simulink model "hrg_5e_tdm_shared_readout_mismatch"  (R2025a)
settings: Solver=FixedStepDiscrete  StartTime=0.0  StopTime=c.duration  FixedStep=c.Ts  RelTol=1e-3
model workspace (MAT data in the model file):
  c.mode = 'tdm_shared'
  c.reuse = 1
  c.continuous = 0
  c.Ts = 1.83823529412e-07
  c.w = 42725.6600888
  c.omega = 0.5
  c.duration = 0.3
  c.B = 0.276990961962
  c.n = 800
  c.adcLatency = 5
  c.logDecimation = 200
  c.p.schema = 'v10.1'
  c.p.synthetic = 1
  c.p.f0 = 6800
  c.p.gamma_intrinsic = 0.712094334814
  c.p.Cs = 6e-10
  c.p.G0 = 1e-10
  c.p.kappa = 1e-06
  c.p.b = 1.1e-06
  c.p.Cds = 0
  c.p.Rs = 1000
  c.p.B = 0.276990961962
  c.p.Omega = 0.5
  c.p.Ts = 1.83823529412e-07
  c.p.Tc = 0.001
  c.p.duration = 0.3
  c.p.charge_target = 1e-11
  c.p.initial_fraction = 1
  c.p.theta0 = 0.4
  c.p.Cf = 1e-10
  c.p.Rf = 1000000000
  c.p.driver_tau = [2e-06; 2e-06]
  c.p.afe_bw = [20000; 20000]
  c.p.detect_matrix = [1  0; 0  1]
  c.p.drive_matrix = [20  0; 0  20]
  c.p.split_hz = 0.05
  c.p.stiffness_axis = 0.37
  c.p.damping_half_difference = 0
  c.p.damping_axis = -0.23
  c.p.adc_span = 2
  c.p.adc_bits = 10
  c.p.dac_span = 1
  c.p.dac_bits = 14
  c.p.vmax = 0.5
  c.p.agc_bw = 10
  c.p.quad_bw = 4
  c.p.pll_gain = 30
  c.p.max_detune = 30
  c.p.virtual_rate = 0
  c.p.virtual_start_min_s = 0.25
  c.p.virtual_settle_fraction = 0.01
  c.p.predict_heading = 1
  c.p.max_heading_rate = 100
  c.p.virtual_validated_limit = 0.2
  c.p.min_amplitude_fraction = 0.02
  c.p.min_linearity = 0.1
  c.p.max_calibration_condition = 100
  c.p.max_frame_age = 0.002
  c.p.calibrate_detection = 1
  c.p.calibrate_drive = 1
  c.p.noise_rms_V = 0
  c.p.noise_seed = 52
  c.p.carrier_hz = 6800
  c.p.Q = 30000
  c.p.pre_gain = 1
  c.p.power_gain = 20
  c.p.aaf_order = 4
  c.p.fs = 5440000
  c.p.bleed_R = 15000
  c.p.reset_tau = 2e-06
  c.p.adc_latency = 5
  c.p.log_decimation = 200
  c.p.adc_noise_rms = 0
  c.p.dac_divisor = 1
  c.p.allow_adc_underclock = 0
  c.p.seed_enabled = 0
  c.p.seed_seconds = 0.03
  c.p.seed_voltage = 0.2
  c.p.cv_mode = 'thx2024'
  c.p.thx_cv_gain = 10000
  c.p.thx_charge_per_input = 1e-06
  c.p.cv_source = 'thx2024'
  c.head.f0_Hz = 6800
  c.head.split_Hz = 0.05
  c.head.Q = 30000
  c.head.parasitic_F = 6e-10
  c.head.f_modes_Hz = [6799.975 6800.025]
  c.head.ringdown_s = 1.4043083214
  c.head.linewidth_Hz = 0.226666666667
  c.head.temperature_model = 'No per-head temperature curve supplied'
  c.head.group_shunt_F = [6e-10; 6e-10; 6e-10; 6e-10]
  c.driveEnd = 800
  c.senseStart = 1200
  c.validStart = 2000
  c.validEnd = 2800
  c.frame = 3200
  c.adcStep = 0.001953125
  c.adcMin = -1
  c.adcMax = 0.998046875
  c.dacStep = 6.103515625e-05
  c.dacMin = -0.5
  c.dacMax = 0.499938964844
  c.minEnergy = 0.0004
  c.minLinearity = 0.1
  c.agc = 62.8318530718
  c.gamma = 0.712094334814
  c.quad = 25.1327412287
  c.forceScale = 3.10732073373
  c.startCommand = [0; 0; 0; 0]
  c.seedCommand = [0; 0; -0.184212198801; -0.0778836684617]
  c.stateCount = 28
  c.pickoff = [0  0  0  0  0  0  0  0  0  0  0  0  0  0  0  0  0  0  0  0  0  0  0  0  0  0  0.1  0; 0  0  0  0  0  0  0  0  0  0  0  0  0  0  0  0  0  0  0  0  0  0  0  0  0  0  0  0.1]
  c.motion = [1  0  0  0  0  0  0  0  0  0  0  0  0  0  0  0  0  0  0  0  0  0  0  0  0  0  0  0; 0  1  0  0  0  0  0  0  0  0  0  0  0  0  0  0  0  0  0  0  0  0  0  0  0  0  0  0]
  c.electrode = [0  0  0  0  0  0  0.000213628300444  0  -0.000213628300444  0  0  0  0  0  0  0  0  0  0  0  0  0  0  0  0  0  0  0; 0  0  0  0  0  0  0  0.000213628300444  0  -0.000213628300444  0  0  0  0  0  0  0  0  0  0  0  0  0  0  0  0  0  0]
  c.cvOutputGain = 10000
  c.Ad = [0.999969157815 1.53962513641e-10 -0.00785385721515 3.93391284853e-08 -5.00204063523e-24 -2.06440054698e-29 7.59751211136e-05 -3.80429463917e-10 -7.59751211136e-05 3.80429463917e-10 0 0 ... (784 elements, 28x28)]
  c.Bd = [2.023325338e-09  5.02385057738e-17; -5.01797463451e-17  2.02332533794e-09; 7.91353351691e-07  2.62536050658e-14; -2.62152067382e-14  7.91353351649e-07; 0.0878143670381  8.50341831335e-36; 7.14438114201e-36  0.0878143670381; 3982.13043431  -2.37899750604e-16; 2.37562374806e-16  3982.13043431; -3982.13043431  2.37899750604e-16; -2.37562374806e-16  -3982.13043431; 0  0; 0  0; 0  0; 0  0; 0  0; 0  0; 0  0; 0  0; 0  0; 0  0; 0  0; 0  0; 0  0; 0  0; 0  0; 0  0; 0  0; 0  0]
  c.Af = [0.999969157815 1.53962513639e-10 -0.007853857215 3.93391284845e-08 0 0 0.00119495988637 -5.96524375398e-09 -0.00119495988637 5.96524375398e-09 0 0 ... (784 elements, 28x28)]
  c.As = [0.999969157815 1.53962513639e-10 -0.00785385721501 3.93391284846e-08 0 0 0.00108910486535 -5.43767539195e-09 -0.00108910486535 5.43767539195e-09 -0.0228351677547 -8.48854209834e-14 ... (784 elements, 28x28)]
  c.x0 = [0.921060994003; 0.389418342309; 0; 0; 0; 0; 0; 0; 0; 0; 0; 0; 0; 0; 0; 0; 0; 0; 0; 0; 0; 0; 0; 0; 0; 0; 0; 0]
  c.detect = [-2.88929518877  0  -12.1098125956  0; 0  -2.88929518877  0  -12.1098125956; 12.1098125956  0  -2.88929518877  0; 0  12.1098125956  0  -2.88929518877]
  c.drive = [0.0249909095414  0  0.00224085346117  0; 0  0.0249909095414  0  0.00224085346117; -0.00224085346117  0  0.0249909095414  0; 0  -0.00224085346117  0  0.0249909095414]
  c.gain_check.drive_pre_V_per_V = 1
  c.gain_check.sense_pre_V_per_V = 1
  c.gain_check.driver_post_gain = 20
  c.gain_check.detector_V_per_normalized_charge = 0.0803230761321
  c.gain_check.electrode_limit_V = 10
  c.gain_check.drive_modal_V_per_command = 39.8546525898
  c.gain_check.drive_condition = 1
  c.gain_check.sense_condition = 1
  c.thx_comparison.saved_Kcvd = 10000
  c.thx_comparison.saved_Kcvs = 100000
  c.thx_comparison.saved_Kcsd = 10000
  c.thx_comparison.saved_Kcss = 100000
  c.thx_comparison.matched_cv_gain = 10000
  c.thx_comparison.piezo_charge_per_input_unit_C = 1e-06
  c.thx_comparison.reuse_scope = 'THX static readout Gain, matched to drive channel source value. Piezo adapter and AAF are external.'
  c.stateRows = {'1:4', '5:6', '7:10', '11:26', '27:28'}
  c.portDriveMap = [1  0; 0  1; -1  0; 0  -1]
  c.portSenseMap = [0.5  0  -0.5  0; 0  0.5  0  -0.5]
  c.portCoupling = [1  0; 0  1; -1  0; 0  -1]
  c.portCapacitance_F = [6e-10  0  0  0; 0  6e-10  0  0; 0  0  6e-10  0; 0  0  0  6e-10]
  c.portShuntCapacitance_F = [6e-10; 6e-10; 6e-10; 6e-10]
  c.groupAngles_deg = [0; 45; 90; 135]
  c.groupNames = {'A', 'B', 'C', 'D'}
  c.commonTerminal = 'COM'
  c.portOptions.group_angles_deg = [0; 45; 90; 135]
  c.portOptions.group_charge_gain = [1; 1; 1; 1]
  c.portOptions.group_capacitance_F = [6e-10; 6e-10; 6e-10; 6e-10]
  c.portOptions.drive_on_resistance_ohm = 10
  c.portCV = [0  0  0  0  0  0  0  0  0  0  0  0  0  0  0  0  0  0  0  0  0  0  0.1  0  0  0  0  0; 0  0  0  0  0  0  0  0  0  0  0  0  0  0  0  0  0  0  0  0  0  0  0  0.1  0  0  0  0; 0  0  0  0  0  0  0  0  0  0  0  0  0  0  0  0  0  0  0  0  0  0  0  0  0.1  0  0  0; 0  0  0  0  0  0  0  0  0  0  0  0  0  0  0  0  0  0  0  0  0  0  0  0  0  0.1  0  0]
  c.readoutAnalogMismatch.readout_channel_gain = [1.01; 0.99]
  c.readoutAnalogMismatch.readout_channel_pole_Hz = [85000; 110000]
  c.readoutAnalogMismatch.readout_calibrate = 0
  c.groupVoltage = [0  0  0  0  0  0  0.000427256600888  0  0  0  0  0  0  0  0  0  0  0  0  0  0  0  0  0  0  0  0  0; 0  0  0  0  0  0  0  0.000427256600888  0  0  0  0  0  0  0  0  0  0  0  0  0  0  0  0  0  0  0  0; 0  0  0  0  0  0  0  0  0.000427256600888  0  0  0  0  0  0  0  0  0  0  0  0  0  0  0  0  0  0  0; 0  0  0  0  0  0  0  0  0  0.000427256600888  0  0  0  0  0  0  0  0  0  0  0  0  0  0  0  0  0  0]
  c.readoutCarrierResponse = [1.00357710652-0.0802861685215i; 0.986231129963-0.0609670153068i]
Description:
  | 6800 Hz whole-angle gyro. Four grouped terminals A/B/C/D relative to COM. See five_config for signed routing and physical assumptions. Native blocks only; trace columns 23:26 are the group terminal voltages.
settings Model: Creator=Administrator  LastModifiedBy=Administrator

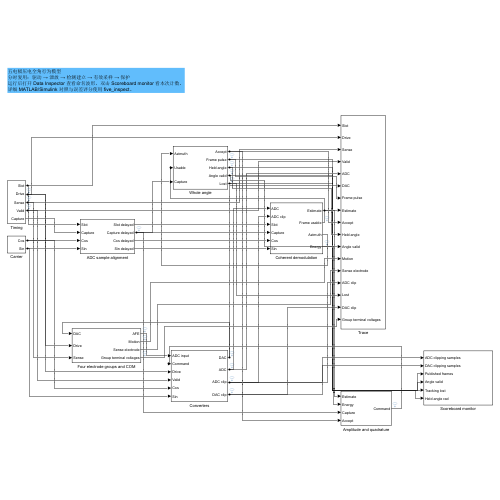
[thumbnail: Simulink's stored preview of the top-level diagram]
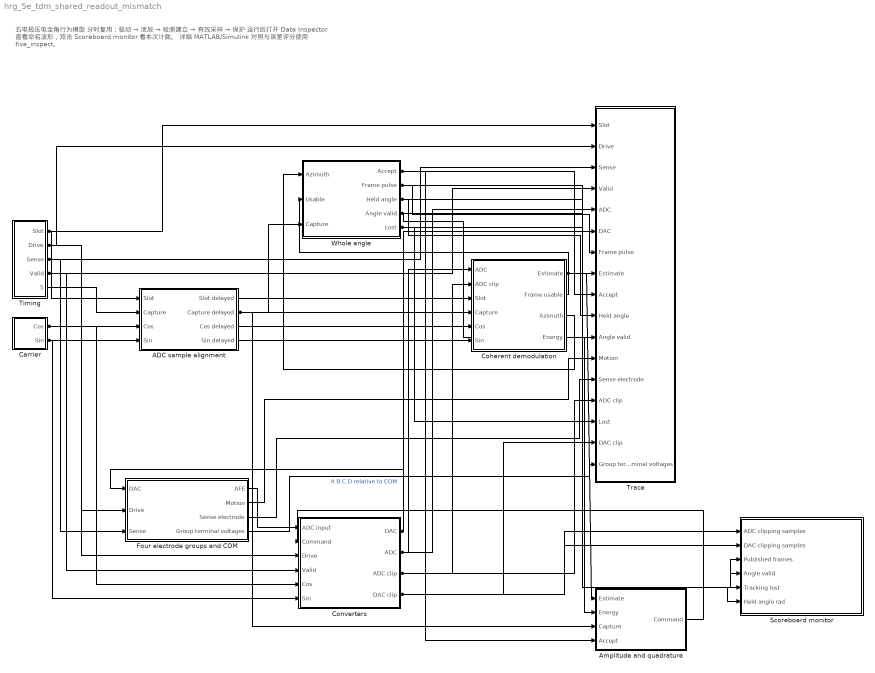
== system hrg_5e_tdm_shared_readout_mismatch ==
  note: 五电极压电全角行为模型
      | 分时复用：驱动 → 泄放 → 检测建立 → 有效采样 → 保护
      | 运行后打开 Data Inspector 查看命名波形，双击 Scoreboard monitor 看本次计数。
      | 详细 MATLAB/Simulink 对照与误差评分使用 five_inspect。
  ADC sample alignment : Subsystem
  Amplitude and quadrature : Subsystem
  Carrier : Subsystem
  Coherent demodulation : Subsystem
  Converters : Subsystem
  Four electrode groups and COM : Subsystem
  Scoreboard monitor : Subsystem
  Timing : Subsystem
  Trace : Subsystem
  Whole angle : Subsystem
  wires:
  Timing/1(Slot) -> Trace/1(Slot), ADC sample alignment/1(Slot)
  Coherent demodulation/4(Energy) -> Amplitude and quadrature/2(Energy)
  Coherent demodulation/1(Estimate) -> Amplitude and quadrature/1(Estimate), Trace/8(Estimate)
  Timing/2(Drive) -> Trace/2(Drive), Converters/3(Drive), Four electrode groups and COM/2(Drive)
  Timing/3(Sense) -> Trace/3(Sense), Four electrode groups and COM/3(Sense)
  Carrier/2(Sin) -> ADC sample alignment/4(Sin), Converters/6(Sin)
  ADC sample alignment/3(Cos delayed) -> Coherent demodulation/5(Cos)
  Carrier/1(Cos) -> Converters/5(Cos), ADC sample alignment/3(Cos)
  Converters/3(ADC clip) -> Trace/14(ADC clip), Coherent demodulation/2(ADC clip), Scoreboard monitor/1(ADC clipping samples)
  Timing/4(Valid) -> Trace/4(Valid), Converters/4(Valid)
  Amplitude and quadrature/1(Command) -> Converters/2(Command)
  ADC sample alignment/4(Sin delayed) -> Coherent demodulation/6(Sin)
  Timing/5(Capture) -> ADC sample alignment/2(Capture)
  ADC sample alignment/1(Slot delayed) -> Coherent demodulation/3(Slot)
  ADC sample alignment/2(Capture delayed) -> Coherent demodulation/4(Capture), Amplitude and quadrature/3(Capture), Whole angle/3(Capture)
  Whole angle/5(Lost) -> Trace/15(Lost), Scoreboard monitor/5(Tracking lost)
  Four electrode groups and COM/1(AFE) -> Converters/1(ADC input)
  Four electrode groups and COM/2(Motion) -> Trace/12(Motion)
  Four electrode groups and COM/3(Sense electrode) -> Trace/13(Sense electrode)
  Four electrode groups and COM/4(Group terminal voltages) -> Trace/17(Group terminal voltages)  "A B C D relative to COM"
  Converters/2(ADC) -> Trace/5(ADC), Coherent demodulation/1(ADC)
  Whole angle/1(Accept) -> Amplitude and quadrature/4(Accept), Trace/9(Accept)
  Whole angle/2(Frame pulse) -> Trace/7(Frame pulse), Scoreboard monitor/3(Published frames)
  Whole angle/3(Held angle) -> Trace/10(Held angle), Scoreboard monitor/6(Held angle rad)
  Whole angle/4(Angle valid) -> Trace/11(Angle valid), Scoreboard monitor/4(Angle valid)
  Converters/1(DAC) -> Four electrode groups and COM/1(DAC), Trace/6(DAC)
  Converters/4(DAC clip) -> Trace/16(DAC clip), Scoreboard monitor/2(DAC clipping samples)
  Coherent demodulation/2(Frame usable) -> Whole angle/2(Usable)
  Coherent demodulation/3(Azimuth) -> Whole angle/1(Azimuth)

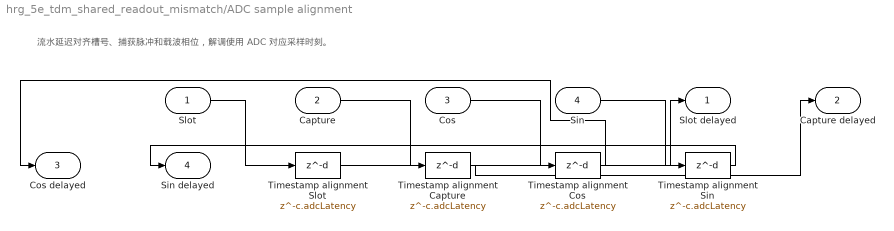
== system hrg_5e_tdm_shared_readout_mismatch/ADC sample alignment ==
  note: 流水延迟对齐槽号、捕获脉冲和载波相位，解调使用 ADC 对应采样时刻。
  Slot : Inport
  Capture : Inport  Port=2
  Cos : Inport  Port=3
  Sin : Inport  Port=4
  Timestamp alignment Capture : Delay  DelayLength=c.adcLatency  InitialCondition=0  SampleTime=c.Ts
  Timestamp alignment Cos : Delay  DelayLength=c.adcLatency  InitialCondition=0  SampleTime=c.Ts
  Timestamp alignment Sin : Delay  DelayLength=c.adcLatency  InitialCondition=0  SampleTime=c.Ts
  Timestamp alignment Slot : Delay  DelayLength=c.adcLatency  InitialCondition=-1  SampleTime=c.Ts
  Slot delayed : Outport
  Capture delayed : Outport  Port=2
  Cos delayed : Outport  Port=3
  Sin delayed : Outport  Port=4
  wires:
  Slot/1 -> Timestamp alignment Slot/1
  Timestamp alignment Slot/1 -> Slot delayed/1
  Capture/1 -> Timestamp alignment Capture/1
  Timestamp alignment Capture/1 -> Capture delayed/1
  Cos/1 -> Timestamp alignment Cos/1
  Timestamp alignment Cos/1 -> Cos delayed/1
  Sin/1 -> Timestamp alignment Sin/1
  Timestamp alignment Sin/1 -> Sin delayed/1

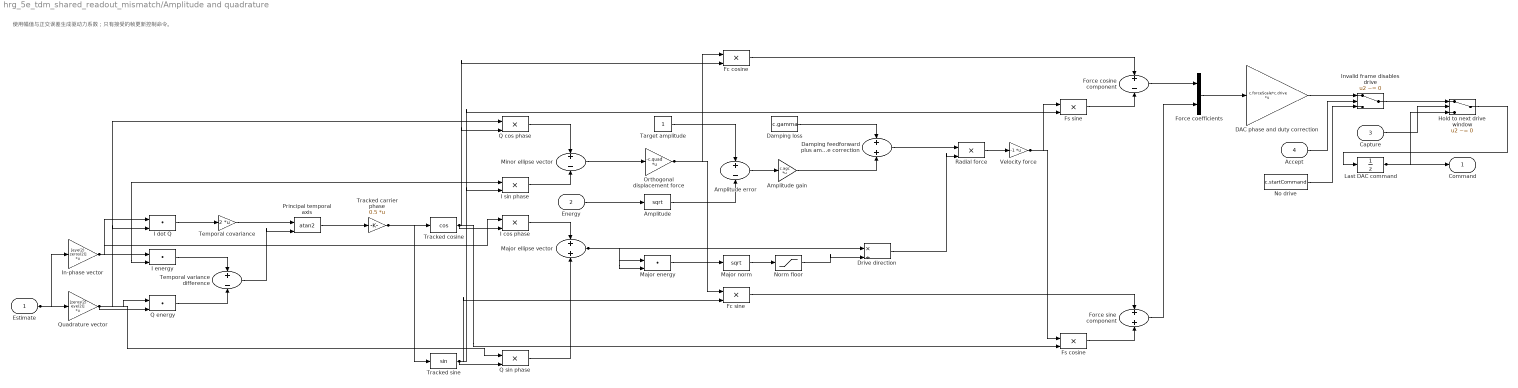
== system hrg_5e_tdm_shared_readout_mismatch/Amplitude and quadrature ==
  note: 使用幅值与正交误差生成驱动力系数；只有接受的帧更新控制命令。
  Estimate : Inport
  Energy : Inport  Port=2
  Capture : Inport  Port=3
  Accept : Inport  Port=4
  Amplitude : Sqrt
  Amplitude error : Sum  Inputs=+-
  Amplitude gain : Gain  Gain=c.agc  Multiplication=Matrix(K*u)
  DAC phase and duty correction : Gain  Gain=c.forceScale*c.drive  Multiplication=Matrix(K*u)
  Damping feedforward plus amplitude correction : Sum
  Damping loss : Constant  Value=c.gamma
  Drive direction : Product  Inputs=*/
  Fc cosine : Product
  Fc sine : Product
  Force coefficients : Mux  Inputs=2
  Force cosine component : Sum  Inputs=+-
  Force sine component : Sum
  Fs cosine : Product
  Fs sine : Product
  Hold to next drive window : Switch  Criteria=u2 ~= 0  SaturateOnIntegerOverflow=off  InputSameDT=off
  I cos phase : Product
  I dot Q : DotProduct  OutDataTypeStr=Inherit: Inherit via internal rule
  I energy : DotProduct  OutDataTypeStr=Inherit: Inherit via internal rule
  I sin phase : Product
  In-phase vector : Gain  Gain=[eye(2) zeros(2)]  Multiplication=Matrix(K*u)
  Invalid frame disables drive : Switch  Criteria=u2 ~= 0  SaturateOnIntegerOverflow=off  InputSameDT=off
  Last DAC command : UnitDelay  InitialCondition=c.startCommand  SampleTime=c.Ts  HasFrameUpgradeWarning=on
  Major ellipse vector : Sum
  Major energy : DotProduct  OutDataTypeStr=Inherit: Inherit via internal rule
  Major norm : Sqrt
  Minor ellipse vector : Sum  Inputs=+-
  No drive : Constant  Value=c.startCommand
  Norm floor : Saturate  UpperLimit=inf  LowerLimit=1e-9
  Orthogonal displacement force : Gain  Gain=-c.quad  Multiplication=Matrix(K*u)
  Principal temporal axis : Trigonometry  Operator=atan2
  Q cos phase : Product
  Q energy : DotProduct  OutDataTypeStr=Inherit: Inherit via internal rule
  Q sin phase : Product
  Quadrature vector : Gain  Gain=[zeros(2) eye(2)]  Multiplication=Matrix(K*u)
  Radial force : Product
  Target amplitude : Constant
  Temporal covariance : Gain  Gain=2  Multiplication=Matrix(K*u)
  Temporal variance difference : Sum  Inputs=+-
  Tracked carrier phase : Gain  Gain=0.5  Multiplication=Matrix(K*u)
  Tracked cosine : Trigonometry  Operator=cos
  Tracked sine : Trigonometry
  Velocity force : Gain  Gain=-1  Multiplication=Matrix(K*u)
  Command : Outport
  wires:
  Estimate/1 -> In-phase vector/1, Quadrature vector/1
  Temporal covariance/1 -> Principal temporal axis/1
  I dot Q/1 -> Temporal covariance/1
  In-phase vector/1 -> I cos phase/1, I sin phase/1, I energy/2, I energy/1, I dot Q/1
  Tracked carrier phase/1 -> Tracked cosine/1, Tracked sine/1
  Temporal variance difference/1 -> Principal temporal axis/2
  Minor ellipse vector/1 -> Orthogonal displacement force/1
  Quadrature vector/1 -> Q sin phase/1, Q cos phase/1, Q energy/1, Q energy/2, I dot Q/2
  I energy/1 -> Temporal variance difference/1
  Q energy/1 -> Temporal variance difference/2
  Principal temporal axis/1 -> Tracked carrier phase/1
  Damping feedforward plus amplitude correction/1 -> Radial force/1
  Tracked cosine/1 -> Fs cosine/2, I cos phase/2, Q cos phase/2, Fc cosine/2
  Tracked sine/1 -> Fs sine/2, I sin phase/2, Q sin phase/2, Fc sine/2
  No drive/1 -> Invalid frame disables drive/3
  Fs cosine/1 -> Force sine component/2
  I cos phase/1 -> Major ellipse vector/1
  Q cos phase/1 -> Minor ellipse vector/1
  I sin phase/1 -> Minor ellipse vector/2
  Q sin phase/1 -> Major ellipse vector/2
  Energy/1 -> Amplitude/1
  DAC phase and duty correction/1 -> Invalid frame disables drive/1
  Major ellipse vector/1 -> Drive direction/1, Major energy/1, Major energy/2
  Target amplitude/1 -> Amplitude error/1
  Orthogonal displacement force/1 -> Fc cosine/1, Fc sine/1
  Amplitude/1 -> Amplitude error/2
  Major energy/1 -> Major norm/1
  Fc cosine/1 -> Force cosine component/1
  Amplitude error/1 -> Amplitude gain/1
  Major norm/1 -> Norm floor/1
  Fc sine/1 -> Force sine component/1
  Damping loss/1 -> Damping feedforward plus amplitude correction/1
  Amplitude gain/1 -> Damping feedforward plus amplitude correction/2
  Norm floor/1 -> Drive direction/2
  Drive direction/1 -> Radial force/2
  Radial force/1 -> Velocity force/1
  Velocity force/1 -> Fs sine/1, Fs cosine/1
  Fs sine/1 -> Force cosine component/2
  Force cosine component/1 -> Force coefficients/1
  Force sine component/1 -> Force coefficients/2
  Force coefficients/1 -> DAC phase and duty correction/1
  Accept/1 -> Invalid frame disables drive/2
  Invalid frame disables drive/1 -> Hold to next drive window/1
  Capture/1 -> Hold to next drive window/2
  Last DAC command/1 -> Hold to next drive window/3, Command/1
  Hold to next drive window/1 -> Last DAC command/1

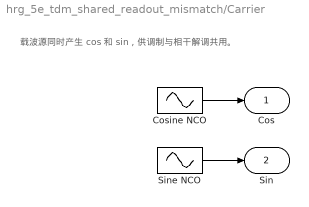
== system hrg_5e_tdm_shared_readout_mismatch/Carrier ==
  note: 载波源同时产生 cos 和 sin，供调制与相干解调共用。
  Cosine NCO : Sin  Frequency=c.w  Phase=pi/2  SampleTime=c.Ts
  Sine NCO : Sin  Frequency=c.w  SampleTime=c.Ts
  Cos : Outport
  Sin : Outport  Port=2
  wires:
  Cosine NCO/1 -> Cos/1
  Sine NCO/1 -> Sin/1

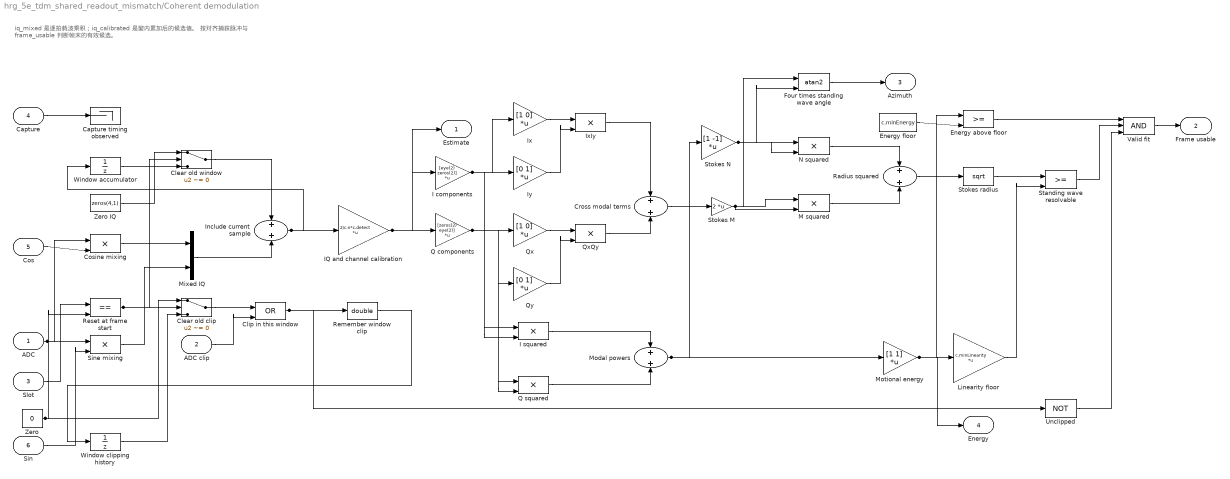
== system hrg_5e_tdm_shared_readout_mismatch/Coherent demodulation ==
  note: iq_mixed 是逐拍载波乘积；iq_calibrated 是窗内累加后的候选值。
      | 按对齐捕获脉冲与 frame_usable 判断帧末的有效候选。
  ADC : Inport
  ADC clip : Inport  Port=2
  Slot : Inport  Port=3
  Capture : Inport  Port=4
  Cos : Inport  Port=5
  Sin : Inport  Port=6
  Capture timing observed : Terminator
  Clear old clip : Switch  Criteria=u2 ~= 0  SaturateOnIntegerOverflow=off  InputSameDT=off
  Clear old window : Switch  Criteria=u2 ~= 0  SaturateOnIntegerOverflow=off  InputSameDT=off
  Clip in this window : Logic  Operator=OR  AllPortsSameDT=off  OutDataTypeStr=boolean
  Cosine mixing : Product
  Cross modal terms : Sum
  Energy above floor : RelationalOperator  OutDataTypeStr=boolean  RndMeth=Simplest  InputSameDT=off
  Energy floor : Constant  Value=c.minEnergy
  Four times standing wave angle : Trigonometry  Operator=atan2
  I components : Gain  Gain=[eye(2) zeros(2)]  Multiplication=Matrix(K*u)
  I squared : Product
  IQ and channel calibration : Gain  Gain=2/c.n*c.detect  Multiplication=Matrix(K*u)
  Include current sample : Sum
  Ix : Gain  Gain=[1 0]  Multiplication=Matrix(K*u)
  IxIy : Product
  Iy : Gain  Gain=[0 1]  Multiplication=Matrix(K*u)
  Linearity floor : Gain  Gain=c.minLinearity  Multiplication=Matrix(K*u)
  M squared : Product
  Mixed IQ : Mux  Inputs=2
  Modal powers : Sum
  Motional energy : Gain  Gain=[1 1]  Multiplication=Matrix(K*u)
  N squared : Product
  Q components : Gain  Gain=[zeros(2) eye(2)]  Multiplication=Matrix(K*u)
  Q squared : Product
  Qx : Gain  Gain=[1 0]  Multiplication=Matrix(K*u)
  QxQy : Product
  Qy : Gain  Gain=[0 1]  Multiplication=Matrix(K*u)
  Radius squared : Sum
  Remember window clip : DataTypeConversion  OutDataTypeStr=double  SaturateOnIntegerOverflow=off  RndMeth=Floor
  Reset at frame start : RelationalOperator  Operator===  OutDataTypeStr=boolean  RndMeth=Simplest  InputSameDT=off
  Sine mixing : Product
  Standing wave resolvable : RelationalOperator  OutDataTypeStr=boolean  RndMeth=Simplest  InputSameDT=off
  Stokes M : Gain  Gain=2  Multiplication=Matrix(K*u)
  Stokes N : Gain  Gain=[1 -1]  Multiplication=Matrix(K*u)
  Stokes radius : Sqrt
  Unclipped : Logic  Operator=NOT  Inputs=1  AllPortsSameDT=off  OutDataTypeStr=boolean
  Valid fit : Logic  Inputs=3  AllPortsSameDT=off  OutDataTypeStr=boolean
  Window accumulator : UnitDelay  InitialCondition=zeros(4,1)  SampleTime=c.Ts  HasFrameUpgradeWarning=on
  Window clipping history : UnitDelay  SampleTime=c.Ts  HasFrameUpgradeWarning=on
  Zero : Constant  Value=0
  Zero IQ : Constant  Value=zeros(4,1)
  Estimate : Outport
  Frame usable : Outport  Port=2
  Azimuth : Outport  Port=3
  Energy : Outport  Port=4
  wires:
  Sin/1 -> Sine mixing/2
  Cos/1 -> Cosine mixing/2
  Modal powers/1 -> Motional energy/1, Stokes N/1
  Sine mixing/1 -> Mixed IQ/2
  Capture/1 -> Capture timing observed/1
  Slot/1 -> Reset at frame start/1
  Stokes N/1 -> Four times standing wave angle/2, N squared/1, N squared/2
  ADC/1 -> Sine mixing/1, Cosine mixing/1
  Zero/1 -> Clear old clip/1, Reset at frame start/2
  Four times standing wave angle/1 -> Azimuth/1
  Window accumulator/1 -> Clear old window/3
  Unclipped/1 -> Valid fit/3
  Ix/1 -> IxIy/1
  Zero IQ/1 -> Clear old window/1
  Cosine mixing/1 -> Mixed IQ/1
  Reset at frame start/1 -> Clear old window/2, Clear old clip/2
  Window clipping history/1 -> Clear old clip/3
  Cross modal terms/1 -> Stokes M/1
  Clear old window/1 -> Include current sample/1
  Mixed IQ/1 -> Include current sample/2
  I components/1 -> I squared/1, I squared/2, Iy/1, Ix/1
  Clear old clip/1 -> Clip in this window/1
  ADC clip/1 -> Clip in this window/2
  Motional energy/1 -> Energy above floor/1, Linearity floor/1, Energy/1
  Include current sample/1 -> Window accumulator/1, IQ and channel calibration/1
  Clip in this window/1 -> Unclipped/1, Remember window clip/1
  IQ and channel calibration/1 -> I components/1, Q components/1, Estimate/1
  Remember window clip/1 -> Window clipping history/1
  Q components/1 -> Q squared/1, Q squared/2, Qx/1, Qy/1
  Iy/1 -> IxIy/2
  Qx/1 -> QxQy/1
  Linearity floor/1 -> Standing wave resolvable/2
  Qy/1 -> QxQy/2
  I squared/1 -> Modal powers/1
  Q squared/1 -> Modal powers/2
  IxIy/1 -> Cross modal terms/1
  QxQy/1 -> Cross modal terms/2
  Valid fit/1 -> Frame usable/1
  Stokes M/1 -> Four times standing wave angle/1, M squared/1, M squared/2
  N squared/1 -> Radius squared/1
  M squared/1 -> Radius squared/2
  Energy floor/1 -> Energy above floor/2
  Radius squared/1 -> Stokes radius/1
  Energy above floor/1 -> Valid fit/1
  Stokes radius/1 -> Standing wave resolvable/1
  Standing wave resolvable/1 -> Valid fit/2

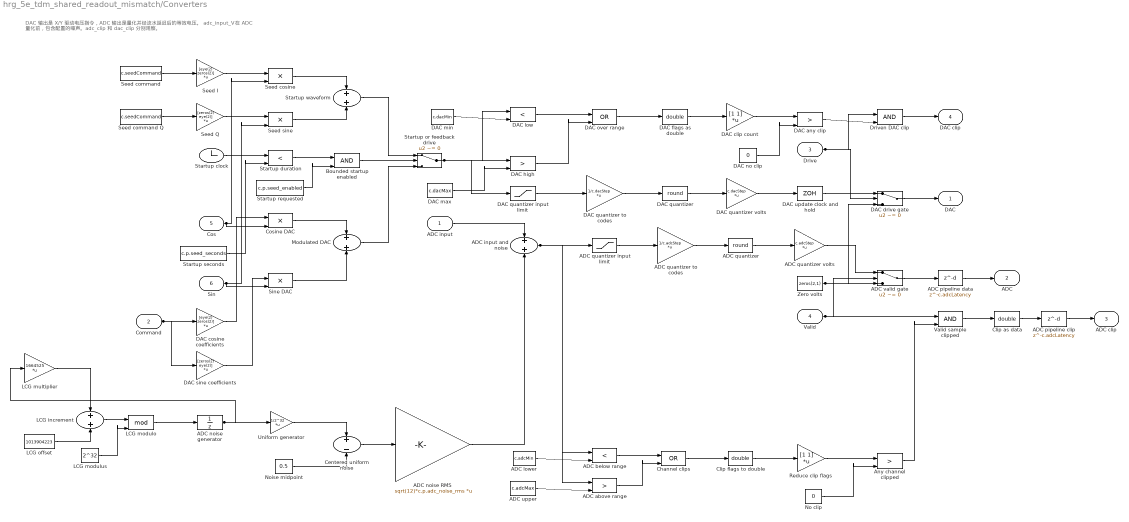
== system hrg_5e_tdm_shared_readout_mismatch/Converters ==
  note: DAC 输出是 X/Y 驱动电压指令，ADC 输出是量化并经流水延迟后的等效电压。
      | adc_input_V 在 ADC 量化前，包含配置的噪声。adc_clip 和 dac_clip 分别观察。
  ADC input : Inport
  Command : Inport  Port=2
  Drive : Inport  Port=3
  Valid : Inport  Port=4
  Cos : Inport  Port=5
  Sin : Inport  Port=6
  ADC above range : RelationalOperator  Operator=>  OutDataTypeStr=boolean  RndMeth=Simplest  InputSameDT=off
  ADC below range : RelationalOperator  Operator=<  OutDataTypeStr=boolean  RndMeth=Simplest  InputSameDT=off
  ADC input and noise : Sum
  ADC lower : Constant  Value=c.adcMin
  ADC noise RMS : Gain  Gain=sqrt(12)*c.p.adc_noise_rms  Multiplication=Matrix(K*u)
  ADC noise generator : UnitDelay  InitialCondition=[c.p.noise_seed;c.p.noise_seed+1]  SampleTime=c.Ts  HasFrameUpgradeWarning=on
  ADC pipeline clip : Delay  DelayLength=c.adcLatency  InitialCondition=0  SampleTime=c.Ts
  ADC pipeline data : Delay  DelayLength=c.adcLatency  InitialCondition=0  SampleTime=c.Ts
  ADC quantizer : Rounding  Operator=round
  ADC quantizer input limit : Saturate  UpperLimit=c.adcMax  LowerLimit=c.adcMin
  ADC quantizer to codes : Gain  Gain=1/c.adcStep  Multiplication=Matrix(K*u)
  ADC quantizer volts : Gain  Gain=c.adcStep  Multiplication=Matrix(K*u)
  ADC upper : Constant  Value=c.adcMax
  ADC valid gate : Switch  Criteria=u2 ~= 0  SaturateOnIntegerOverflow=off  InputSameDT=off
  Any channel clipped : RelationalOperator  Operator=>  OutDataTypeStr=boolean  RndMeth=Simplest  InputSameDT=off
  Bounded startup enabled : Logic  AllPortsSameDT=off  OutDataTypeStr=boolean
  Centered uniform noise : Sum  Inputs=+-
  Channel clips : Logic  Operator=OR  AllPortsSameDT=off  OutDataTypeStr=boolean
  Clip as data : DataTypeConversion  OutDataTypeStr=double  SaturateOnIntegerOverflow=off  RndMeth=Floor
  Clip flags to double : DataTypeConversion  OutDataTypeStr=double  SaturateOnIntegerOverflow=off  RndMeth=Floor
  Cosine DAC : Product
  DAC any clip : RelationalOperator  Operator=>  OutDataTypeStr=boolean  RndMeth=Simplest  InputSameDT=off
  DAC clip count : Gain  Gain=[1 1]  Multiplication=Matrix(K*u)
  DAC cosine coefficients : Gain  Gain=[eye(2) zeros(2)]  Multiplication=Matrix(K*u)
  DAC drive gate : Switch  Criteria=u2 ~= 0  SaturateOnIntegerOverflow=off  InputSameDT=off
  DAC flags as double : DataTypeConversion  OutDataTypeStr=double  SaturateOnIntegerOverflow=off  RndMeth=Floor
  DAC high : RelationalOperator  Operator=>  OutDataTypeStr=boolean  RndMeth=Simplest  InputSameDT=off
  DAC low : RelationalOperator  Operator=<  OutDataTypeStr=boolean  RndMeth=Simplest  InputSameDT=off
  DAC max : Constant  Value=c.dacMax
  DAC min : Constant  Value=c.dacMin
  DAC no clip : Constant  Value=0
  DAC over range : Logic  Operator=OR  AllPortsSameDT=off  OutDataTypeStr=boolean
  DAC quantizer : Rounding  Operator=round
  DAC quantizer input limit : Saturate  UpperLimit=c.dacMax  LowerLimit=c.dacMin
  DAC quantizer to codes : Gain  Gain=1/c.dacStep  Multiplication=Matrix(K*u)
  DAC quantizer volts : Gain  Gain=c.dacStep  Multiplication=Matrix(K*u)
  DAC sine coefficients : Gain  Gain=[zeros(2) eye(2)]  Multiplication=Matrix(K*u)
  DAC update clock and hold : ZeroOrderHold  SampleTime=c.Ts*c.p.dac_divisor
  Driven DAC clip : Logic  AllPortsSameDT=off  OutDataTypeStr=boolean
  LCG increment : Sum
  LCG modulo : Math  Operator=mod
  LCG modulus : Constant  Value=2^32
  LCG multiplier : Gain  Gain=1664525  Multiplication=Matrix(K*u)
  LCG offset : Constant  Value=1013904223
  Modulated DAC : Sum
  No clip : Constant  Value=0
  Noise midpoint : Constant  Value=0.5
  Reduce clip flags : Gain  Gain=[1 1]  Multiplication=Matrix(K*u)
  Seed I : Gain  Gain=[eye(2) zeros(2)]  Multiplication=Matrix(K*u)
  Seed Q : Gain  Gain=[zeros(2) eye(2)]  Multiplication=Matrix(K*u)
  Seed command : Constant  Value=c.seedCommand
  Seed command Q : Constant  Value=c.seedCommand
  Seed cosine : Product
  Seed sine : Product
  Sine DAC : Product
  Startup clock : Clock
  Startup duration : RelationalOperator  Operator=<  OutDataTypeStr=boolean  RndMeth=Simplest  InputSameDT=off
  Startup or feedback drive : Switch  Criteria=u2 ~= 0  SaturateOnIntegerOverflow=off  InputSameDT=off
  Startup requested : Constant  Value=c.p.seed_enabled
  Startup seconds : Constant  Value=c.p.seed_seconds
  Startup waveform : Sum
  Uniform generator : Gain  Gain=1/2^32  Multiplication=Matrix(K*u)
  Valid sample clipped : Logic  AllPortsSameDT=off  OutDataTypeStr=boolean
  Zero volts : Constant  Value=zeros(2,1)
  DAC : Outport
  ADC : Outport  Port=2
  ADC clip : Outport  Port=3
  DAC clip : Outport  Port=4
  wires:
  Seed command/1 -> Seed I/1
  Seed cosine/1 -> Startup waveform/1
  ADC quantizer volts/1 -> ADC valid gate/1
  Startup requested/1 -> Bounded startup enabled/2
  LCG multiplier/1 -> LCG increment/1
  Channel clips/1 -> Clip flags to double/1
  Startup or feedback drive/1 -> DAC quantizer input limit/1, DAC low/1, DAC high/1
  LCG modulus/1 -> LCG modulo/2
  LCG offset/1 -> LCG increment/2
  Reduce clip flags/1 -> Any channel clipped/1
  Cos/1 -> Cosine DAC/2, Seed cosine/2
  LCG increment/1 -> LCG modulo/1
  Bounded startup enabled/1 -> Startup or feedback drive/2
  ADC below range/1 -> Channel clips/1
  Seed command Q/1 -> Seed Q/1
  LCG modulo/1 -> ADC noise generator/1
  Command/1 -> DAC sine coefficients/1, DAC cosine coefficients/1
  ADC input/1 -> ADC input and noise/1
  Seed I/1 -> Seed cosine/1
  Seed Q/1 -> Seed sine/1
  Startup clock/1 -> Startup duration/1
  Startup seconds/1 -> Startup duration/2
  Sin/1 -> Sine DAC/2, Seed sine/2
  ADC quantizer/1 -> ADC quantizer volts/1
  DAC cosine coefficients/1 -> Cosine DAC/1
  DAC sine coefficients/1 -> Sine DAC/1
  DAC min/1 -> DAC low/2
  ADC noise generator/1 -> LCG multiplier/1, Uniform generator/1
  Seed sine/1 -> Startup waveform/2
  ADC quantizer input limit/1 -> ADC quantizer to codes/1
  Startup duration/1 -> Bounded startup enabled/1
  Cosine DAC/1 -> Modulated DAC/1
  No clip/1 -> Any channel clipped/2
  Sine DAC/1 -> Modulated DAC/2
  DAC quantizer volts/1 -> DAC update clock and hold/1
  ADC pipeline data/1 -> ADC/1
  DAC flags as double/1 -> DAC clip count/1
  ADC above range/1 -> Channel clips/2
  Uniform generator/1 -> Centered uniform noise/1
  ADC quantizer to codes/1 -> ADC quantizer/1
  Noise midpoint/1 -> Centered uniform noise/2
  Startup waveform/1 -> Startup or feedback drive/1
  ADC noise RMS/1 -> ADC input and noise/2
  Modulated DAC/1 -> Startup or feedback drive/3
  Centered uniform noise/1 -> ADC noise RMS/1
  DAC max/1 -> DAC high/2
  DAC low/1 -> DAC over range/1
  DAC high/1 -> DAC over range/2
  DAC clip count/1 -> DAC any clip/1
  DAC quantizer input limit/1 -> DAC quantizer to codes/1
  ADC input and noise/1 -> ADC below range/1, ADC quantizer input limit/1, ADC above range/1
  ADC lower/1 -> ADC below range/2
  Zero volts/1 -> DAC drive gate/3, ADC valid gate/3
  Drive/1 -> DAC drive gate/2, Driven DAC clip/1
  ADC upper/1 -> ADC above range/2
  DAC over range/1 -> DAC flags as double/1
  DAC quantizer to codes/1 -> DAC quantizer/1
  DAC quantizer/1 -> DAC quantizer volts/1
  DAC no clip/1 -> DAC any clip/2
  Clip flags to double/1 -> Reduce clip flags/1
  DAC any clip/1 -> Driven DAC clip/2
  DAC update clock and hold/1 -> DAC drive gate/1
  Driven DAC clip/1 -> DAC clip/1
  Valid/1 -> Valid sample clipped/1, ADC valid gate/2
  DAC drive gate/1 -> DAC/1
  ADC valid gate/1 -> ADC pipeline data/1
  Any channel clipped/1 -> Valid sample clipped/2
  Valid sample clipped/1 -> Clip as data/1
  Clip as data/1 -> ADC pipeline clip/1
  ADC pipeline clip/1 -> ADC clip/1

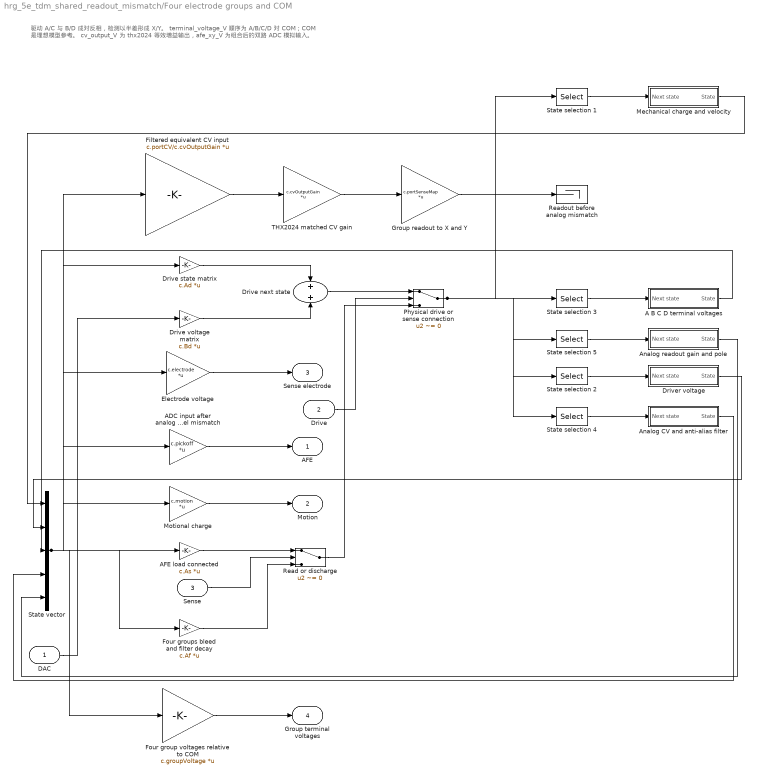
== system hrg_5e_tdm_shared_readout_mismatch/Four electrode groups and COM ==
  note: 驱动 A/C 与 B/D 成对反相，检测以半差形成 X/Y。
      | terminal_voltage_V 顺序为 A/B/C/D 对 COM；COM 是理想模型参考。
      | cv_output_V 为 thx2024 等效增益输出，afe_xy_V 为组合后的双路 ADC 模拟输入。
  DAC : Inport
  Drive : Inport  Port=2
  Sense : Inport  Port=3
  A B C D terminal voltages : Subsystem
  ADC input after analog channel mismatch : Gain  Gain=c.pickoff  Multiplication=Matrix(K*u)
  AFE load connected : Gain  Gain=c.As  Multiplication=Matrix(K*u)
  Analog CV and anti-alias filter : Subsystem
  Analog readout gain and pole : Subsystem
  Drive next state : Sum
  Drive state matrix : Gain  Gain=c.Ad  Multiplication=Matrix(K*u)
  Drive voltage matrix : Gain  Gain=c.Bd  Multiplication=Matrix(K*u)
  Driver voltage : Subsystem
  Electrode voltage : Gain  Gain=c.electrode  Multiplication=Matrix(K*u)
  Filtered equivalent CV input : Gain  Gain=c.portCV/c.cvOutputGain  Multiplication=Matrix(K*u)
  Four group voltages relative to COM : Gain  Gain=c.groupVoltage  Multiplication=Matrix(K*u)
  Four groups bleed and filter decay : Gain  Gain=c.Af  Multiplication=Matrix(K*u)
  Group readout to X and Y : Gain  Gain=c.portSenseMap  Multiplication=Matrix(K*u)
  Mechanical charge and velocity : Subsystem
  Motional charge : Gain  Gain=c.motion  Multiplication=Matrix(K*u)
  Physical drive or sense connection : Switch  Criteria=u2 ~= 0  SaturateOnIntegerOverflow=off  InputSameDT=off
  Read or discharge : Switch  Criteria=u2 ~= 0  SaturateOnIntegerOverflow=off  InputSameDT=off
  Readout before analog mismatch : Terminator
  State selection 1 : Selector  InputPortWidth=28  IndexOptions=Index vector (dialog)  Indices=1:4  OutputSizes=1
  State selection 2 : Selector  InputPortWidth=28  IndexOptions=Index vector (dialog)  Indices=5:6  OutputSizes=1
  State selection 3 : Selector  InputPortWidth=28  IndexOptions=Index vector (dialog)  Indices=7:10  OutputSizes=1
  State selection 4 : Selector  InputPortWidth=28  IndexOptions=Index vector (dialog)  Indices=11:26  OutputSizes=1
  State selection 5 : Selector  InputPortWidth=28  IndexOptions=Index vector (dialog)  Indices=27:28  OutputSizes=1
  State vector : Mux  Inputs=5
  THX2024 matched CV gain : Gain  Gain=c.cvOutputGain  Multiplication=Matrix(K*u)
  AFE : Outport
  Motion : Outport  Port=2
  Sense electrode : Outport  Port=3
  Group terminal voltages : Outport  Port=4
  wires:
  AFE load connected/1 -> Read or discharge/1
  ADC input after analog channel mismatch/1 -> AFE/1
  State vector/1 -> Drive state matrix/1, Filtered equivalent CV input/1, ADC input after analog channel mismatch/1, Motional charge/1, AFE load connected/1, Electrode voltage/1, Four group voltages relative to COM/1, Four groups bleed and filter decay/1
  Electrode voltage/1 -> Sense electrode/1
  Drive state matrix/1 -> Drive next state/1
  Sense/1 -> Read or discharge/2
  DAC/1 -> Drive voltage matrix/1
  Filtered equivalent CV input/1 -> THX2024 matched CV gain/1
  Drive voltage matrix/1 -> Drive next state/2
  Drive/1 -> Physical drive or sense connection/2
  Motional charge/1 -> Motion/1
  Four groups bleed and filter decay/1 -> Read or discharge/3
  Four group voltages relative to COM/1 -> Group terminal voltages/1
  THX2024 matched CV gain/1 -> Group readout to X and Y/1
  Group readout to X and Y/1 -> Readout before analog mismatch/1
  Drive next state/1 -> Physical drive or sense connection/1
  Read or discharge/1 -> Physical drive or sense connection/3
  Physical drive or sense connection/1 -> State selection 1/1, State selection 2/1, State selection 3/1, State selection 4/1, State selection 5/1
  State selection 1/1 -> Mechanical charge and velocity/1(Next state)
  State selection 3/1 -> A B C D terminal voltages/1(Next state)
  State selection 5/1 -> Analog readout gain and pole/1(Next state)
  A B C D terminal voltages/1(State) -> State vector/3
  State selection 2/1 -> Driver voltage/1(Next state)
  State selection 4/1 -> Analog CV and anti-alias filter/1(Next state)
  Mechanical charge and velocity/1(State) -> State vector/1
  Analog readout gain and pole/1(State) -> State vector/5
  Analog CV and anti-alias filter/1(State) -> State vector/4
  Driver voltage/1(State) -> State vector/2

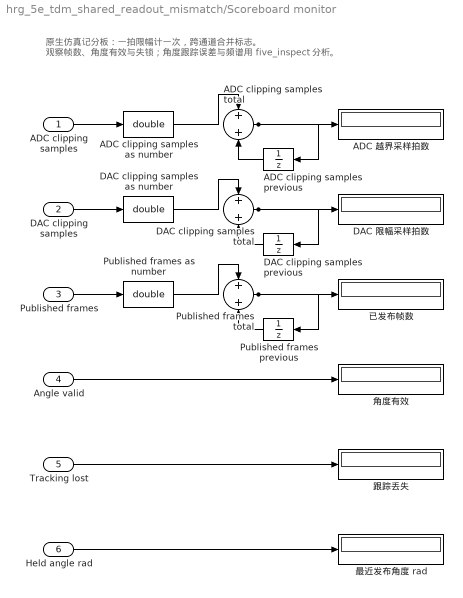
== system hrg_5e_tdm_shared_readout_mismatch/Scoreboard monitor ==
  note: 原生仿真记分板：一拍限幅计一次，跨通道合并标志。
      | 观察帧数、角度有效与失锁；角度跟踪误差与频谱用 five_inspect 分析。
  ADC clipping samples : Inport
  DAC clipping samples : Inport  Port=2
  Published frames : Inport  Port=3
  Angle valid : Inport  Port=4
  Tracking lost : Inport  Port=5
  Held angle rad : Inport  Port=6
  ADC clipping samples as number : DataTypeConversion  OutDataTypeStr=double  SaturateOnIntegerOverflow=off  RndMeth=Floor
  ADC clipping samples previous : UnitDelay  SampleTime=c.Ts  HasFrameUpgradeWarning=on
  ADC clipping samples total : Sum
  ADC 越界采样拍数 : Display
  DAC clipping samples as number : DataTypeConversion  OutDataTypeStr=double  SaturateOnIntegerOverflow=off  RndMeth=Floor
  DAC clipping samples previous : UnitDelay  SampleTime=c.Ts  HasFrameUpgradeWarning=on
  DAC clipping samples total : Sum
  DAC 限幅采样拍数 : Display
  Published frames as number : DataTypeConversion  OutDataTypeStr=double  SaturateOnIntegerOverflow=off  RndMeth=Floor
  Published frames previous : UnitDelay  SampleTime=c.Ts  HasFrameUpgradeWarning=on
  Published frames total : Sum
  已发布帧数 : Display
  最近发布角度 rad : Display
  角度有效 : Display
  跟踪丢失 : Display
  wires:
  ADC clipping samples/1 -> ADC clipping samples as number/1
  ADC clipping samples as number/1 -> ADC clipping samples total/1
  ADC clipping samples total/1 -> ADC clipping samples previous/1, ADC 越界采样拍数/1
  ADC clipping samples previous/1 -> ADC clipping samples total/2
  DAC clipping samples/1 -> DAC clipping samples as number/1
  DAC clipping samples as number/1 -> DAC clipping samples total/1
  DAC clipping samples total/1 -> DAC clipping samples previous/1, DAC 限幅采样拍数/1
  DAC clipping samples previous/1 -> DAC clipping samples total/2
  Published frames/1 -> Published frames as number/1
  Published frames as number/1 -> Published frames total/1
  Published frames total/1 -> Published frames previous/1, 已发布帧数/1
  Published frames previous/1 -> Published frames total/2
  Angle valid/1 -> 角度有效/1
  Tracking lost/1 -> 跟踪丢失/1
  Held angle rad/1 -> 最近发布角度 rad/1

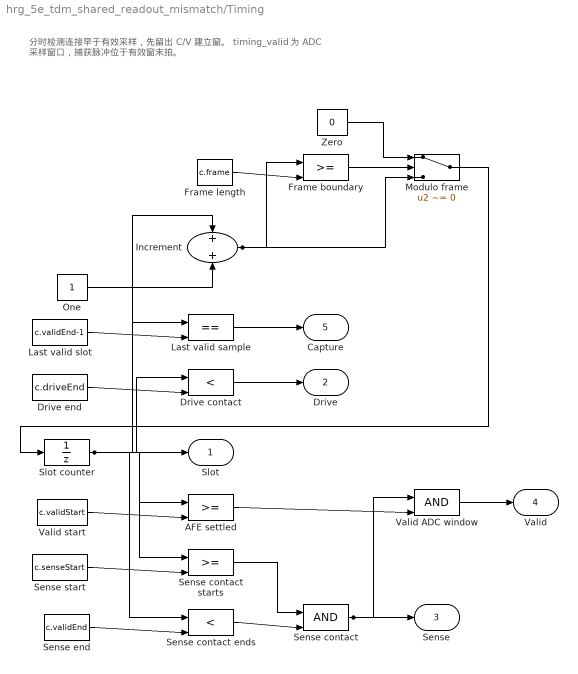
== system hrg_5e_tdm_shared_readout_mismatch/Timing ==
  note: 分时检测连接早于有效采样，先留出 C/V 建立窗。
      | timing_valid 为 ADC 采样窗口，捕获脉冲位于有效窗末拍。
  AFE settled : RelationalOperator  OutDataTypeStr=boolean  RndMeth=Simplest  InputSameDT=off
  Drive contact : RelationalOperator  Operator=<  OutDataTypeStr=boolean  RndMeth=Simplest  InputSameDT=off
  Drive end : Constant  Value=c.driveEnd
  Frame boundary : RelationalOperator  OutDataTypeStr=boolean  RndMeth=Simplest  InputSameDT=off
  Frame length : Constant  Value=c.frame
  Increment : Sum
  Last valid sample : RelationalOperator  Operator===  OutDataTypeStr=boolean  RndMeth=Simplest  InputSameDT=off
  Last valid slot : Constant  Value=c.validEnd-1
  Modulo frame : Switch  Criteria=u2 ~= 0  SaturateOnIntegerOverflow=off  InputSameDT=off
  One : Constant
  Sense contact : Logic  AllPortsSameDT=off  OutDataTypeStr=boolean
  Sense contact ends : RelationalOperator  Operator=<  OutDataTypeStr=boolean  RndMeth=Simplest  InputSameDT=off
  Sense contact starts : RelationalOperator  OutDataTypeStr=boolean  RndMeth=Simplest  InputSameDT=off
  Sense end : Constant  Value=c.validEnd
  Sense start : Constant  Value=c.senseStart
  Slot counter : UnitDelay  SampleTime=c.Ts  HasFrameUpgradeWarning=on
  Valid ADC window : Logic  AllPortsSameDT=off  OutDataTypeStr=boolean
  Valid start : Constant  Value=c.validStart
  Zero : Constant  Value=0
  Slot : Outport
  Drive : Outport  Port=2
  Sense : Outport  Port=3
  Valid : Outport  Port=4
  Capture : Outport  Port=5
  wires:
  One/1 -> Increment/2
  Last valid slot/1 -> Last valid sample/2
  Drive end/1 -> Drive contact/2
  Frame length/1 -> Frame boundary/2
  Slot counter/1 -> Drive contact/1, Sense contact starts/1, Increment/1, Last valid sample/1, Slot/1, AFE settled/1, Sense contact ends/1
  Valid start/1 -> AFE settled/2
  Last valid sample/1 -> Capture/1
  Sense end/1 -> Sense contact ends/2
  Sense start/1 -> Sense contact starts/2
  Increment/1 -> Modulo frame/3, Frame boundary/1
  Drive contact/1 -> Drive/1
  AFE settled/1 -> Valid ADC window/2
  Sense contact starts/1 -> Sense contact/1
  Sense contact ends/1 -> Sense contact/2
  Zero/1 -> Modulo frame/1
  Frame boundary/1 -> Modulo frame/2
  Sense contact/1 -> Valid ADC window/1, Sense/1
  Valid ADC window/1 -> Valid/1
  Modulo frame/1 -> Slot counter/1

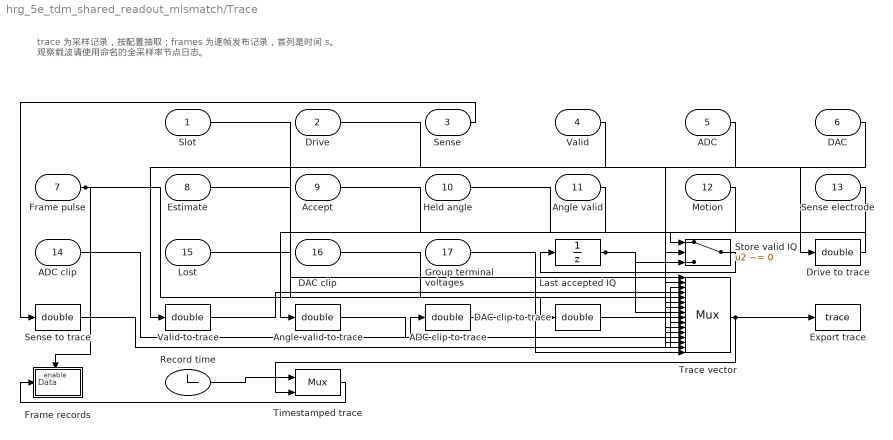
== system hrg_5e_tdm_shared_readout_mismatch/Trace ==
  note: trace 为采样记录，按配置抽取；frames 为逐帧发布记录，首列是时间 s。
      | 观察载波请使用命名的全采样率节点日志。
  Slot : Inport
  Drive : Inport  Port=2
  Sense : Inport  Port=3
  Valid : Inport  Port=4
  ADC : Inport  Port=5
  DAC : Inport  Port=6
  Frame pulse : Inport  Port=7
  Estimate : Inport  Port=8
  Accept : Inport  Port=9
  Held angle : Inport  Port=10
  Angle valid : Inport  Port=11
  Motion : Inport  Port=12
  Sense electrode : Inport  Port=13
  ADC clip : Inport  Port=14
  Lost : Inport  Port=15
  DAC clip : Inport  Port=16
  Group terminal voltages : Inport  Port=17
  ADC clip to trace : DataTypeConversion  OutDataTypeStr=double  SaturateOnIntegerOverflow=off  RndMeth=Floor
  Angle valid to trace : DataTypeConversion  OutDataTypeStr=double  SaturateOnIntegerOverflow=off  RndMeth=Floor
  DAC clip to trace : DataTypeConversion  OutDataTypeStr=double  SaturateOnIntegerOverflow=off  RndMeth=Floor
  Drive to trace : DataTypeConversion  OutDataTypeStr=double  SaturateOnIntegerOverflow=off  RndMeth=Floor
  Export trace : ToWorkspace  VariableName=trace  SampleTime=-1
      settings: Decimation=c.logDecimation
  Frame records : Subsystem
  Last accepted IQ : UnitDelay  InitialCondition=zeros(4,1)  SampleTime=c.Ts  HasFrameUpgradeWarning=on
  Record time : Clock
  Sense to trace : DataTypeConversion  OutDataTypeStr=double  SaturateOnIntegerOverflow=off  RndMeth=Floor
  Store valid IQ : Switch  Criteria=u2 ~= 0  SaturateOnIntegerOverflow=off  InputSameDT=off
  Timestamped trace : Mux  Inputs=2
  Trace vector : Mux  Inputs=16
  Valid to trace : DataTypeConversion  OutDataTypeStr=double  SaturateOnIntegerOverflow=off  RndMeth=Floor
  wires:
  Estimate/1 -> Store valid IQ/1
  Accept/1 -> Store valid IQ/2
  Last accepted IQ/1 -> Store valid IQ/3, Trace vector/8
  Store valid IQ/1 -> Last accepted IQ/1
  Drive/1 -> Drive to trace/1
  Sense/1 -> Sense to trace/1
  Valid/1 -> Valid to trace/1
  Angle valid/1 -> Angle valid to trace/1
  ADC clip/1 -> ADC clip to trace/1
  DAC clip/1 -> DAC clip to trace/1
  Slot/1 -> Trace vector/1
  Drive to trace/1 -> Trace vector/2
  Sense to trace/1 -> Trace vector/3
  Valid to trace/1 -> Trace vector/4
  ADC/1 -> Trace vector/5
  DAC/1 -> Trace vector/6
  Frame pulse/1 -> Trace vector/7, Frame records/Enable
  Held angle/1 -> Trace vector/9
  Angle valid to trace/1 -> Trace vector/10
  Motion/1 -> Trace vector/11
  Sense electrode/1 -> Trace vector/12
  ADC clip to trace/1 -> Trace vector/13
  Lost/1 -> Trace vector/14
  DAC clip to trace/1 -> Trace vector/15
  Group terminal voltages/1 -> Trace vector/16
  Trace vector/1 -> Export trace/1, Timestamped trace/2
  Record time/1 -> Timestamped trace/1
  Timestamped trace/1 -> Frame records/1(Data)

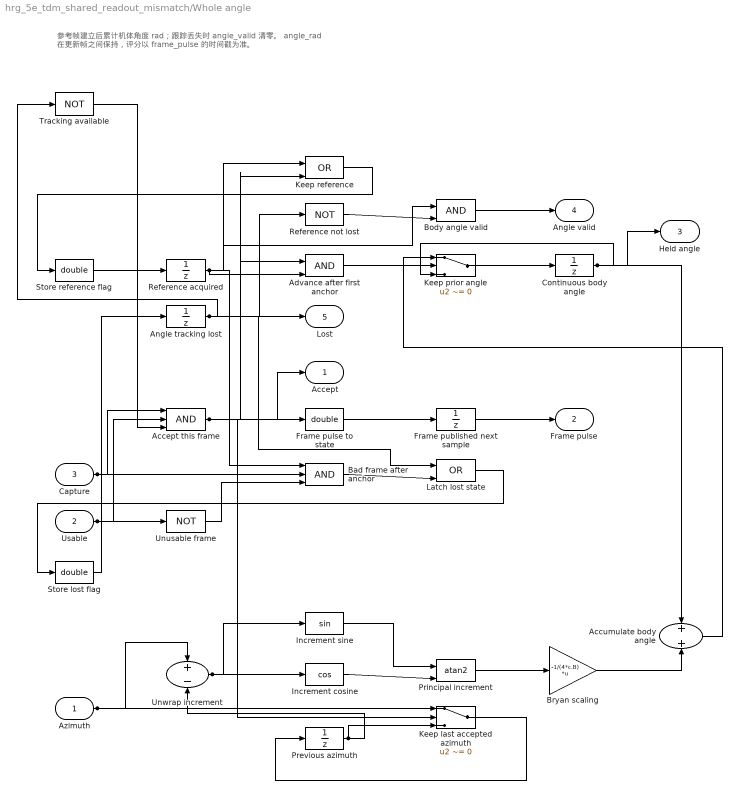
== system hrg_5e_tdm_shared_readout_mismatch/Whole angle ==
  note: 参考帧建立后累计机体角度 rad；跟踪丢失时 angle_valid 清零。
      | angle_rad 在更新帧之间保持，评分以 frame_pulse 的时间戳为准。
  Azimuth : Inport
  Usable : Inport  Port=2
  Capture : Inport  Port=3
  Accept this frame : Logic  Inputs=3  AllPortsSameDT=off  OutDataTypeStr=boolean
  Accumulate body angle : Sum
  Advance after first anchor : Logic  AllPortsSameDT=off  OutDataTypeStr=boolean
  Angle tracking lost : UnitDelay  SampleTime=c.Ts  HasFrameUpgradeWarning=on
  Bad frame after anchor : Logic  Inputs=3  AllPortsSameDT=off  OutDataTypeStr=boolean
  Body angle valid : Logic  AllPortsSameDT=off  OutDataTypeStr=boolean
  Bryan scaling : Gain  Gain=-1/(4*c.B)  Multiplication=Matrix(K*u)
  Continuous body angle : UnitDelay  SampleTime=c.Ts  HasFrameUpgradeWarning=on
  Frame published next sample : UnitDelay  SampleTime=c.Ts  HasFrameUpgradeWarning=on
  Frame pulse to state : DataTypeConversion  OutDataTypeStr=double  SaturateOnIntegerOverflow=off  RndMeth=Floor
  Increment cosine : Trigonometry  Operator=cos
  Increment sine : Trigonometry
  Keep last accepted azimuth : Switch  Criteria=u2 ~= 0  SaturateOnIntegerOverflow=off  InputSameDT=off
  Keep prior angle : Switch  Criteria=u2 ~= 0  SaturateOnIntegerOverflow=off  InputSameDT=off
  Keep reference : Logic  Operator=OR  AllPortsSameDT=off  OutDataTypeStr=boolean
  Latch lost state : Logic  Operator=OR  AllPortsSameDT=off  OutDataTypeStr=boolean
  Previous azimuth : UnitDelay  SampleTime=c.Ts  HasFrameUpgradeWarning=on
  Principal increment : Trigonometry  Operator=atan2
  Reference acquired : UnitDelay  SampleTime=c.Ts  HasFrameUpgradeWarning=on
  Reference not lost : Logic  Operator=NOT  Inputs=1  AllPortsSameDT=off  OutDataTypeStr=boolean
  Store lost flag : DataTypeConversion  OutDataTypeStr=double  SaturateOnIntegerOverflow=off  RndMeth=Floor
  Store reference flag : DataTypeConversion  OutDataTypeStr=double  SaturateOnIntegerOverflow=off  RndMeth=Floor
  Tracking available : Logic  Operator=NOT  Inputs=1  AllPortsSameDT=off  OutDataTypeStr=boolean
  Unusable frame : Logic  Operator=NOT  Inputs=1  AllPortsSameDT=off  OutDataTypeStr=boolean
  Unwrap increment : Sum  Inputs=+-
  Accept : Outport
  Frame pulse : Outport  Port=2
  Held angle : Outport  Port=3
  Angle valid : Outport  Port=4
  Lost : Outport  Port=5
  wires:
  Tracking available/1 -> Accept this frame/3
  Store reference flag/1 -> Reference acquired/1
  Angle tracking lost/1 -> Tracking available/1, Latch lost state/1, Lost/1, Reference not lost/1
  Capture/1 -> Bad frame after anchor/2, Accept this frame/1
  Usable/1 -> Accept this frame/2, Unusable frame/1
  Reference acquired/1 -> Body angle valid/1, Keep reference/1, Bad frame after anchor/1, Advance after first anchor/2
  Store lost flag/1 -> Angle tracking lost/1
  Azimuth/1 -> Unwrap increment/1, Keep last accepted azimuth/1
  Accept this frame/1 -> Keep reference/2, Frame pulse to state/1, Keep last accepted azimuth/2, Advance after first anchor/1, Accept/1
  Unusable frame/1 -> Bad frame after anchor/3
  Unwrap increment/1 -> Increment sine/1, Increment cosine/1
  Keep reference/1 -> Store reference flag/1
  Reference not lost/1 -> Body angle valid/2
  Advance after first anchor/1 -> Keep prior angle/2
  Frame pulse to state/1 -> Frame published next sample/1
  Bad frame after anchor/1 -> Latch lost state/2
  Increment sine/1 -> Principal increment/1
  Increment cosine/1 -> Principal increment/2
  Previous azimuth/1 -> Unwrap increment/2, Keep last accepted azimuth/3
  Body angle valid/1 -> Angle valid/1
  Keep prior angle/1 -> Continuous body angle/1
  Frame published next sample/1 -> Frame pulse/1
  Latch lost state/1 -> Store lost flag/1
  Principal increment/1 -> Bryan scaling/1
  Keep last accepted azimuth/1 -> Previous azimuth/1
  Continuous body angle/1 -> Accumulate body angle/1, Held angle/1, Keep prior angle/3
  Bryan scaling/1 -> Accumulate body angle/2
  Accumulate body angle/1 -> Keep prior angle/1

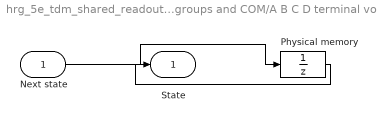
== system hrg_5e_tdm_shared_readout_mismatch/Four electrode groups and COM/A B C D terminal voltages ==
  Next state : Inport
  Physical memory : UnitDelay  InitialCondition=c.x0(7:10)  SampleTime=c.Ts  HasFrameUpgradeWarning=on
  State : Outport
  wires:
  Next state/1 -> Physical memory/1
  Physical memory/1 -> State/1

== system hrg_5e_tdm_shared_readout_mismatch/Four electrode groups and COM/Analog CV and anti-alias filter ==
  Next state : Inport
  Physical memory : UnitDelay  InitialCondition=c.x0(11:26)  SampleTime=c.Ts  HasFrameUpgradeWarning=on
  State : Outport
  wires:
  Next state/1 -> Physical memory/1
  Physical memory/1 -> State/1

== system hrg_5e_tdm_shared_readout_mismatch/Four electrode groups and COM/Analog readout gain and pole ==
  Next state : Inport
  Physical memory : UnitDelay  InitialCondition=c.x0(27:28)  SampleTime=c.Ts  HasFrameUpgradeWarning=on
  State : Outport
  wires:
  Next state/1 -> Physical memory/1
  Physical memory/1 -> State/1

== system hrg_5e_tdm_shared_readout_mismatch/Four electrode groups and COM/Driver voltage ==
  Next state : Inport
  Physical memory : UnitDelay  InitialCondition=c.x0(5:6)  SampleTime=c.Ts  HasFrameUpgradeWarning=on
  State : Outport
  wires:
  Next state/1 -> Physical memory/1
  Physical memory/1 -> State/1

== system hrg_5e_tdm_shared_readout_mismatch/Four electrode groups and COM/Mechanical charge and velocity ==
  Next state : Inport
  Physical memory : UnitDelay  InitialCondition=c.x0(1:4)  SampleTime=c.Ts  HasFrameUpgradeWarning=on
  State : Outport
  wires:
  Next state/1 -> Physical memory/1
  Physical memory/1 -> State/1

== system hrg_5e_tdm_shared_readout_mismatch/Trace/Frame records ==
  Data : Inport
  Enable : EnablePort
  Export frames : ToWorkspace  VariableName=frames  SampleTime=-1
  wires:
  Data/1 -> Export frames/1
